simulink model "Controlador_LQR_lim"  (R2026b)
settings: Solver=FixedStepDiscrete  StopTime=inf  FixedStep=Ts  EnableMultiTasking=on
InitFcn:
  | init_BOOT
values from neighbouring files (symbols this model uses):
  AW_activo = 1    [init_BOOT.m]
  DeltaD_max = Duty_max - D0    (= 32)    [init_BOOT.m]
  DeltaD_min = Duty_min - D0    (= -5)    [init_BOOT.m]
  Ki_LQR = K_LQR(3)    [init_BOOT.m]
  Ku_LQR = K_LQR(2)    [init_BOOT.m]
  Kx_LQR = K_LQR(1)    [init_BOOT.m]
  Ts = evalin('base', 'Ts')    [ejecutar_PIL.m]    (also in init_BOOT.m = 0.00025; prueba_independencia_PIL.m)
undefined symbols (not defined in the file or in its folder): DiscIntNeverNeededParam
settings Model: SILPILModeSetting=veronly  Creator=Usuario  LastModifiedBy=matia
settings SolverCC: AutoInsertRateTranBlk=on
settings DataIOCC: SaveOutput=off  SaveTime=off
settings OptimizationCC: DifferentSizesBufferReuse=on  EfficientTunableParamExpr=on  EnhancedBackFolding=on  MaxStackSize=64  OptimizationCustomize=off  OptimizeBlockOrder=speed  PassReuseOutputArgsAs=Individual arguments
settings DebuggingCC: ParameterTunabilityLossMsg=error
settings HardwareCC: ProdHWDeviceType=Atmel->AVR  ProdLargestAtomicFloat=None
settings ModelReferenceCC: PropagateVarSize=During execution
settings SFSimCC: MATLABDynamicMemAlloc=off
settings RTWCC: BuildConfiguration=Faster Runs  Description=Embedded Coder  HardwareBoard=Arduino Mega 2560  SystemTargetFile=ert.tlc  TLCOptions=-aInlineSetEventsForThisBaseRateFcn=TLC_FALSE -aSuppressMultiTaskScheduler=TLC_FALSE -aRateBasedStepFcn=1  TemplateMakefile=ert_default_tmf  Toolchain=Arduino AVR
settings CodeAppCC: ForceParamTrailComments=on  IgnoreCustomStorageClasses=off  InsertBlockDesc=on  OperatorAnnotations=on  SFDataObjDesc=on  SimulinkDataObjDesc=on
settings ERTTargetCC: CodeInterfacePackaging=Reusable function  ExtModeAutomaticAllocSize=off  ExtModeIntrfLevel=Level2 - Open  ExtModeMexFile=ext_xcp  ExtModeStaticAlloc=on  RootIOFormat=Structure reference  SupportContinuousTime=on  SupportVariableSizeSignals=on

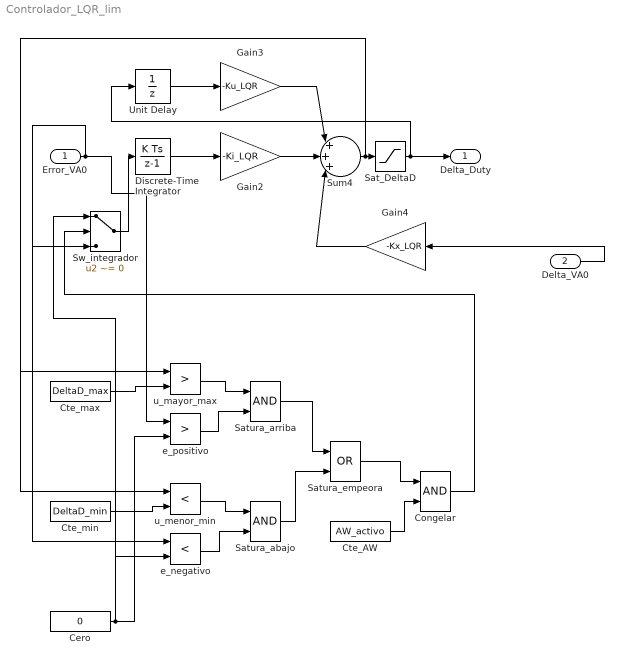
== system Controlador_LQR_lim ==
  Error_VA0 : Inport  OutDataTypeStr=single  PortDimensions=1  SampleTime=[0.00025000000000000001,0]
  Delta_VA0 : Inport  Port=2  OutDataTypeStr=single  PortDimensions=1  SampleTime=[0.00025000000000000001,0]
  Cero : Constant  Value=0  OutDataTypeStr=single
  Congelar : Logic  AllPortsSameDT=off  OutDataTypeStr=boolean
  Cte_AW : Constant  Value=AW_activo  OutDataTypeStr=boolean
  Cte_max : Constant  Value=DeltaD_max  OutDataTypeStr=single
  Cte_min : Constant  Value=DeltaD_min  OutDataTypeStr=single
  Discrete-Time Integrator : DiscreteIntegrator  SampleTime=Ts  OutDataTypeStr=single  ICPrevOutput=DiscIntNeverNeededParam  ICPrevScaledInput=DiscIntNeverNeededParam
  Gain2 : Gain  Gain=-Ki_LQR  OutDataTypeStr=Inherit: Same as input  ParamDataTypeStr=Inherit: Same as input
  Gain3 : Gain  Gain=-Ku_LQR  OutDataTypeStr=Inherit: Same as input  ParamDataTypeStr=Inherit: Same as input
  Gain4 : Gain  Gain=-Kx_LQR  OutDataTypeStr=Inherit: Same as input  ParamDataTypeStr=Inherit: Same as input
  Sat_DeltaD : Saturate  UpperLimit=DeltaD_max  LowerLimit=DeltaD_min
  Satura_abajo : Logic  AllPortsSameDT=off  OutDataTypeStr=boolean
  Satura_arriba : Logic  AllPortsSameDT=off  OutDataTypeStr=boolean
  Satura_empeora : Logic  Operator=OR  AllPortsSameDT=off  OutDataTypeStr=boolean
  Sum4 : Sum  Inputs=|+++|  OutDataTypeStr=single
  Sw_integrador : Switch  Criteria=u2 ~= 0  SaturateOnIntegerOverflow=off  InputSameDT=off
  Unit Delay : UnitDelay  SampleTime=Ts
  e_negativo : RelationalOperator  Operator=<  OutDataTypeStr=boolean  RndMeth=Simplest  InputSameDT=off
  e_positivo : RelationalOperator  Operator=>  OutDataTypeStr=boolean  RndMeth=Simplest  InputSameDT=off
  u_mayor_max : RelationalOperator  Operator=>  OutDataTypeStr=boolean  RndMeth=Simplest  InputSameDT=off
  u_menor_min : RelationalOperator  Operator=<  OutDataTypeStr=boolean  RndMeth=Simplest  InputSameDT=off
  Delta_Duty : Outport  OutDataTypeStr=single  PortDimensions=1  SampleTime=[0.00025000000000000001,0]
  wires:
  Unit Delay/1 -> Gain3/1
  Discrete-Time Integrator/1 -> Gain2/1
  Delta_VA0/1 -> Gain4/1
  Gain3/1 -> Sum4/1
  Gain2/1 -> Sum4/2
  Gain4/1 -> Sum4/3
  Sum4/1 -> Sat_DeltaD/1, u_mayor_max/1, u_menor_min/1
  Sat_DeltaD/1 -> Delta_Duty/1, Unit Delay/1
  Cte_max/1 -> u_mayor_max/2
  Error_VA0/1 -> e_positivo/1, e_negativo/1, Sw_integrador/3
  Cero/1 -> e_positivo/2, e_negativo/2, Sw_integrador/1
  Cte_min/1 -> u_menor_min/2
  u_mayor_max/1 -> Satura_arriba/1
  e_positivo/1 -> Satura_arriba/2
  u_menor_min/1 -> Satura_abajo/1
  e_negativo/1 -> Satura_abajo/2
  Satura_arriba/1 -> Satura_empeora/1
  Satura_abajo/1 -> Satura_empeora/2
  Satura_empeora/1 -> Congelar/1
  Cte_AW/1 -> Congelar/2
  Congelar/1 -> Sw_integrador/2
  Sw_integrador/1 -> Discrete-Time Integrator/1
